simulink subsystem "PIDController"  (R2026a)
settings: Solver=VariableStepAuto
undefined symbols (not defined in the file): PID
settings Model: Creator=Dell  LastModifiedBy=Carlos Fabian

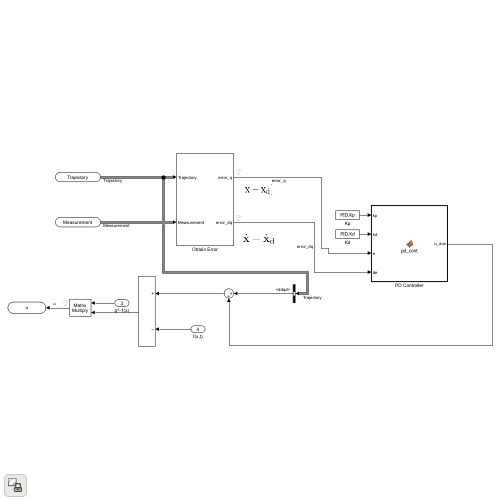
[thumbnail: Simulink's stored preview of the top-level diagram]
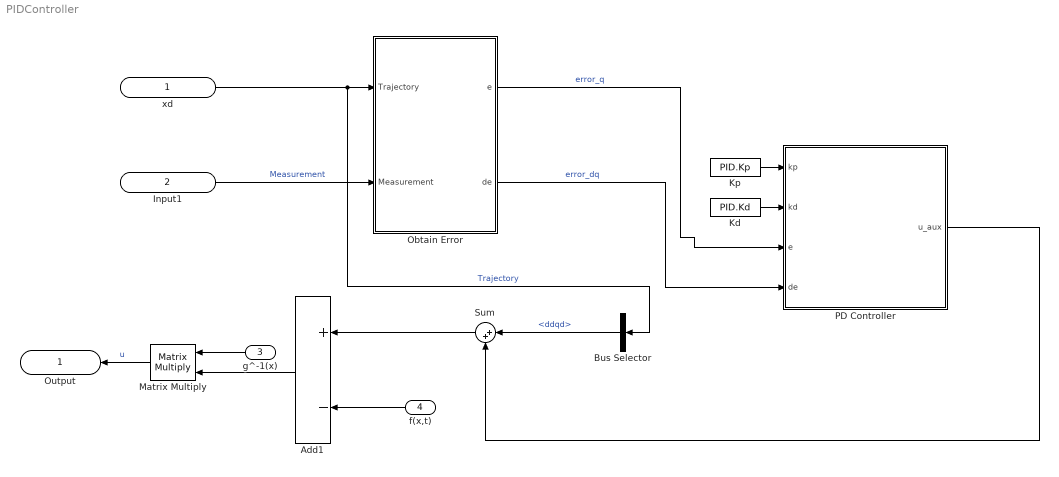
== system PIDController ==
  xd : Inport
  Input1 : Inport  Port=2
  g^-1(x) : Inport  Port=3
  f(x,t) : Inport  Port=4
  Add1 : Sum  Inputs=+-
  Bus Selector : BusSelector  OutputSignals=ddqd
  Kd : Constant  Value=PID.Kd
  Kp : Constant  Value=PID.Kp
  Matrix Multiply : Product  Multiplication=Matrix(*)
  Obtain Error : Subsystem
  PD Controller : MATLAB Function  TreatAsAtomicUnit=on
  Sum : Sum  Inputs=|++
  Output : Outport
  wires:
  Input1/1 -> Obtain Error/2(Measurement)  "Measurement"
  xd/1 -> Bus Selector/1, Obtain Error/1(Trajectory)  "Trajectory"
  Obtain Error/2(de) -> PD Controller/4(de)  "error_dq"
  Obtain Error/1(e) -> PD Controller/3(e)  "error_q"
  f(x,t)/1 -> Add1/2
  g^-1(x)/1 -> Matrix Multiply/1
  Add1/1 -> Matrix Multiply/2
  Matrix Multiply/1 -> Output/1  "u"
  Kp/1 -> PD Controller/1(kp)
  Kd/1 -> PD Controller/2(kd)
  PD Controller/1(u_aux) -> Sum/2
  Bus Selector/1 -> Sum/1  "<ddqd>"
  Sum/1 -> Add1/1

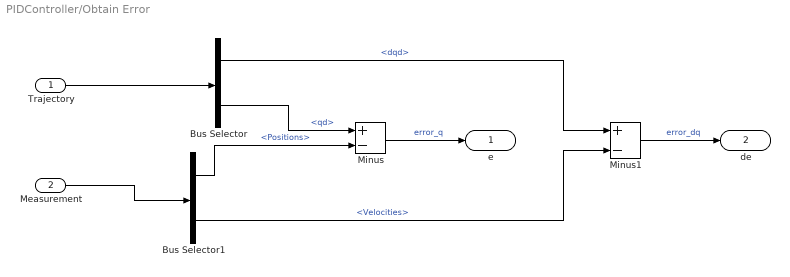
== system PIDController/Obtain Error ==
  Trajectory : Inport
  Measurement : Inport  Port=2
  Bus Selector : BusSelector  OutputSignals=dqd,qd
  Bus Selector1 : BusSelector  OutputSignals=Positions,Velocities
  Minus : Sum  Inputs=+-
  Minus1 : Sum  Inputs=+-
  e : Outport
  de : Outport  Port=2
  wires:
  Minus1/1 -> de/1  "error_dq"
  Minus/1 -> e/1  "error_q"
  Bus Selector/2 -> Minus/1  "<qd>"
  Bus Selector/1 -> Minus1/1  "<dqd>"
  Trajectory/1 -> Bus Selector/1
  Measurement/1 -> Bus Selector1/1
  Bus Selector1/2 -> Minus1/2  "<Velocities>"
  Bus Selector1/1 -> Minus/2  "<Positions>"

== matlab function PIDController/PD Controller ==
  data: kp input; kd input; u_aux output; e input; de input
function u_aux = pd_cont(kp, kd, e, de)


kp_m = [kp(1) 0       0     0     0       0     0     0;
        0     kp(2)   0     0     0       0     0     0;
        0     0       kp(3) 0     0       0     0     0;
        0     0       0     kp(4) 0       0     0     0;
        0     0       0     0     kp(5)   0     0     0;
        0     0       0     0     0       kp(6) 0     0;
        0     0       0     0     0       0     kp(7) 0;
        0     0       0     0     0       0     0     kp(8)];

kd_m = [kd(1) 0       0     0     0       0     0     0;
        0     kd(2)   0     0     0       0     0     0;
        0     0       kd(3) 0     0       0     0     0;
        0     0       0     kd(4) 0       0     0     0;
        0     0       0     0     kd(5)   0     0     0;
        0     0       0     0     0       kd(6) 0     0;
        0     0       0     0     0       0     kd(7) 0;
        0     0       0     0     0       0     0     kd(8)];


%v = ddP + kp_m * e + kd_m * de;
u_aux = kp_m * e + kd_m * de;
%v = ddP;

end
